simulink model "SLX_Morgado"  (R2026b)
settings: Solver=VariableStepAuto
InitFcn:
  | init_val
values from neighbouring files (symbols this model uses):
  fric_coeffs = [0 0.6 0.9 1 0.95 0.75 0.4 0.1]    [init_val.m]
  g = 9.81    [init_val.m]
  j = 1    [init_val.m]
  m = 200    [init_val.m]
  r = 0.3    [init_val.m]
  slip = [0 0.05 0.1 0.15 0.2 0.3 0.5 1]    [init_val.m]
  v_initial = 25    [init_val.m]
settings Model: Creator=zanas  LastModifiedBy=zanas

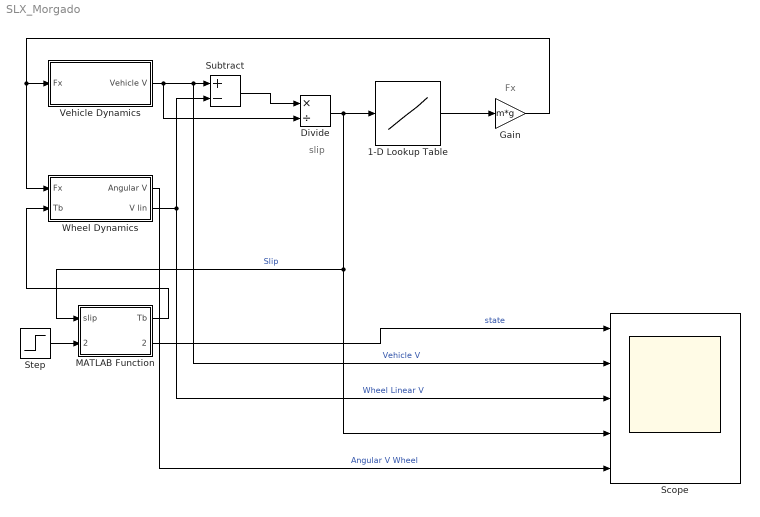
== system SLX_Morgado ==
  note: Fx
  note: slip
  1-D Lookup Table : Lookup_n-D  NumberOfTableDimensions=1  BreakpointsForDimension1=slip  Table=fric_coeffs  InternalRulePriority=Speed  RndMeth=Simplest
  Divide : Product  Inputs=*/
  Gain : Gain  Gain=m*g
  MATLAB Function : MATLAB Function  TreatAsAtomicUnit=on
  Scope : Scope  NumInputPorts=5
      settings: ActiveDisplayYMinimum=-57882.089740993135  ActiveDisplayYMaximum=8845.28329830704
  Step : Step  SampleTime=0
  Subtract : Sum  Inputs=+-
  Vehicle Dynamics : Subsystem
  Wheel Dynamics : Subsystem
  wires:
  Wheel Dynamics/2(V lin) -> Scope/3, Subtract/2  "Wheel Linear V"
  Vehicle Dynamics/1(Vehicle V) -> Scope/2, Subtract/1, Divide/2  "Vehicle V"
  Subtract/1 -> Divide/1
  Divide/1 -> Scope/4, MATLAB Function/1(slip), 1-D Lookup Table/1  "Slip"
  1-D Lookup Table/1 -> Gain/1
  Gain/1 -> Wheel Dynamics/1(Fx), Vehicle Dynamics/1(Fx)
  MATLAB Function/1(Tb) -> Wheel Dynamics/2(Tb)
  Step/1 -> MATLAB Function/2(braking)
  MATLAB Function/2(state_out) -> Scope/1  "state"
  Wheel Dynamics/1(Angular V) -> Scope/5  "Angular V Wheel"

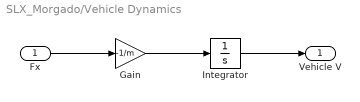
== system SLX_Morgado/Vehicle Dynamics ==
  Fx : Inport
  Gain : Gain  Gain=-1/m
  Integrator : Integrator  InitialCondition=v_initial
  Vehicle V : Outport
  wires:
  Fx/1 -> Gain/1
  Gain/1 -> Integrator/1
  Integrator/1 -> Vehicle V/1

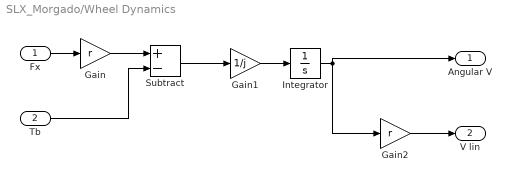
== system SLX_Morgado/Wheel Dynamics ==
  Fx : Inport
  Tb : Inport  Port=2
  Gain : Gain  Gain=r
  Gain1 : Gain  Gain=1/j
  Gain2 : Gain  Gain=r
  Integrator : Integrator  InitialCondition=v_initial/r
  Subtract : Sum  Inputs=+-
  Angular V : Outport
  V lin : Outport  Port=2
  wires:
  Fx/1 -> Gain/1
  Gain/1 -> Subtract/1
  Tb/1 -> Subtract/2
  Subtract/1 -> Gain1/1
  Gain1/1 -> Integrator/1
  Integrator/1 -> Gain2/1, Angular V/1
  Gain2/1 -> V lin/1

== matlab function SLX_Morgado/MATLAB Function ==
  settings: updateMethod=DISCRETE
  data: slip input; Tb output; state_out output; braking input
function [Tb, state_out] = fcn(slip, braking)
% the variable is persistent to remember the state inbetween simulation steps
persistent state;
% starts as inactive which is 1
if isempty(state)
    state = 1; 
end

Tb = 0;
state_out = 1;

if braking == 0
    state = 1; %Inactive
elseif state == 1 && braking > 0
    state = 2; % Regular braking
elseif state == 2 && slip > 0.15
    state = 3; %ABS is turned on
elseif state == 3 && slip < 0.10
    state = 2; %Regular braking
end

switch state
    case 1 %Inactive
        Tb = 0;
        state_out = 1;
    case 2 %Regular braking
        Tb = 800;
        state_out = 2;
    case 3 %ABS is turned on
        Tb = 200;
        state_out = 3;
end
end
